simulink model "MPPT_4x4_grp"  (R2025b)
settings: Solver=ode23t  StartTime=0.0  StopTime=Tstop  MaxStep=1e-4  RelTol=1e-3
model workspace (MAT data in the model file):
  Cin = 0.00022
  Cin_esr = 0.05
  Cout = 0.00047
  G_tau = 0.001
  Gsched = [0 1000 1000 1000 1000 1000 1000 1000 1000 1000 1000 1000 ... (49 elements, 1x49)]
  L = 0.00015
  RL = 0.01
  Rc = 0.05
  Rload = 10
  Tlog = 0.0005
  Tstop = 2
  byp_Goff = 4.4e-06
  byp_Ron = 0.012
  byp_Vf = 0.37
  mppt : object (value not decoded)
  pv_EG = 1.11
  pv_Ir0 = 1000
  pv_Isc = 9.11
  pv_Ncell = 72
  pv_Ngrp = 24
  pv_Rs = 0.00441
  pv_T = 25
  pv_TIPH1 = 0.0005
  pv_TRS1 = 0
  pv_TXIS1 = 6.41
  pv_Tmeas = 25
  pv_Voc = 0.636111111111
  pv_n = 1
  sens : object (value not decoded)
symbols that are objects in the model workspace (value not decoded): mppt, sens
libraries: ee_lib x97, nesl_utility x53, fl_lib x6
(part 4 of 4)

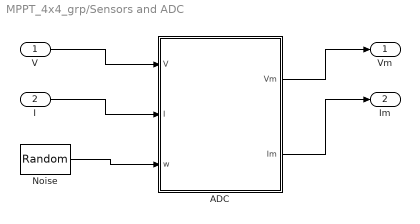
== system MPPT_4x4_grp/Sensors and ADC ==
  V : Inport
  I : Inport  Port=2
  ADC : MATLAB Function  TreatAsAtomicUnit=on
  Noise : RandomNumber  Mean=zeros(1,4)  Variance=ones(1,4)  Seed=sens.seed + (0:3)  SampleTime=mppt.Tc
  Vm : Outport
  Im : Outport  Port=2
  wires:
  V/1 -> ADC/1(V)
  I/1 -> ADC/2(I)
  Noise/1 -> ADC/3(w)
  ADC/1(Vm) -> Vm/1
  ADC/2(Im) -> Im/1

== matlab function MPPT_4x4_grp/Sensors and ADC/ADC ==
  settings: updateMethod=DISCRETE  sampleTime=mppt.Tc
  data: V input; Vm output; I input; w input; Im output; sens parameter
function [Vm, Im] = ADC(V, I, w, sens)
% One call per control sample. The model is in sensor_adc.m.
[Vm, Im] = sensor_adc(V, I, w, sens);

== matlab function MPPT_4x4_grp/Controller/MPPT ==
  settings: updateMethod=DISCRETE  sampleTime=mppt.Tc
  data: Vpv input; D output; Ipv input; Vm output; Im output; ph output; np output; mppt parameter
function [D, Vm, Im, ph, np] = MPPT(Vpv, Ipv, mppt)
% One call per control sample. The algorithm is in mppt_controller.m.
[D, Vm, Im, ph, np] = mppt_controller(Vpv, Ipv, mppt);
